simulink model "Lat_kinematics_Simul"  (R2022b)
settings: Solver=FixedStepAuto  StartTime=0.0  StopTime=tend  FixedStep=0.001  RelTol=1e-3
values from neighbouring files (symbols this model uses):
  lf = 1.4    [Lat_Dynamics_Simul_initialize.m]    (also in Lat_kinematics_Simul_initialize.m)
  lr = 1.6    [Lat_Dynamics_Simul_initialize.m]    (also in Lat_kinematics_Simul_initialize.m)
libraries: robotmobilelib x1
settings Model: Creator=LDW  LastModifiedBy=lego0

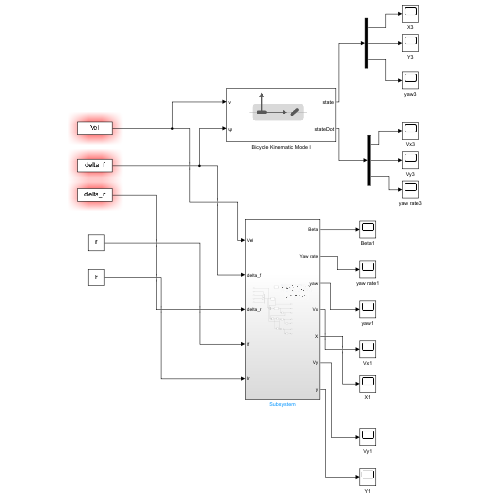
[thumbnail: Simulink's stored preview of the top-level diagram]
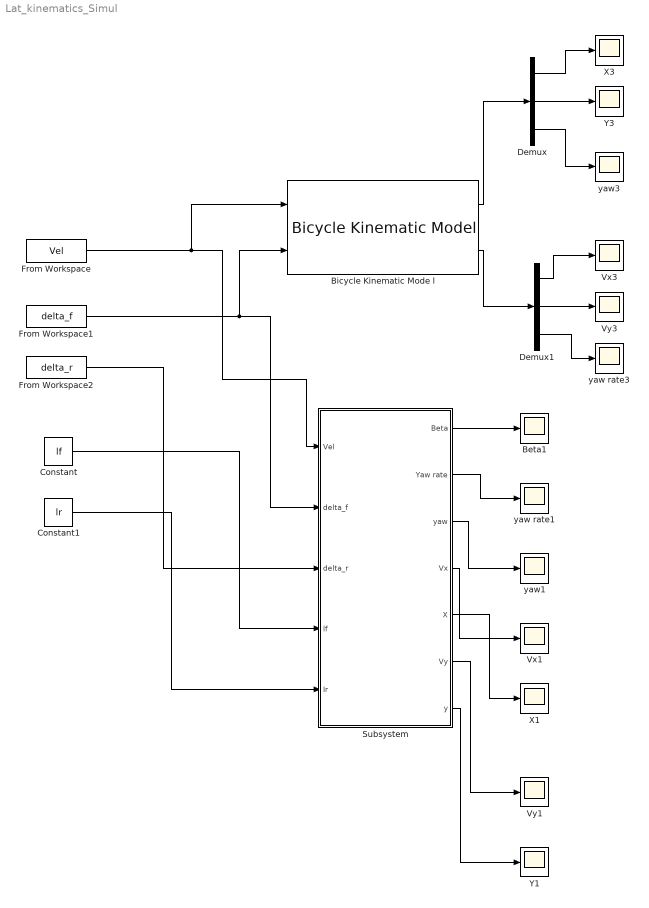
== system Lat_kinematics_Simul ==
  Beta1 : Scope
  Bicycle Kinematic Mode l : robotmobilelib/Bicycle Kinematic Model  VehicleInputs=Vehicle Speed & Steering Angle  WheelBase=3  VehicleSpeedRange=[-inf inf]  MaxSteeringAngle=pi/4  InitialState=[0; 0; 0]  SimulateUsing=Interpreted execution
  Constant : Constant  Value=lf
  Constant1 : Constant  Value=lr
  Demux : Demux  Outputs=3
  Demux1 : Demux  Outputs=3
  From Workspace : FromWorkspace  VariableName=Vel
  From Workspace1 : FromWorkspace  VariableName=delta_f
  From Workspace2 : FromWorkspace  VariableName=delta_r
  Subsystem : Subsystem
  Vx1 : Scope
  Vx3 : Scope
  Vy1 : Scope
  Vy3 : Scope
  X1 : Scope
  X3 : Scope
  Y1 : Scope
  Y3 : Scope
  yaw rate1 : Scope
  yaw rate3 : Scope
  yaw1 : Scope
  yaw3 : Scope
  wires:
  From Workspace/1 -> Subsystem/1(Vel), Bicycle Kinematic Mode l/1
  From Workspace1/1 -> Subsystem/2(delta_f), Bicycle Kinematic Mode l/2
  Bicycle Kinematic Mode l/1 -> Demux/1
  Bicycle Kinematic Mode l/2 -> Demux1/1
  Demux/3 -> yaw3/1
  Demux1/3 -> yaw rate3/1
  Demux1/2 -> Vy3/1
  Demux1/1 -> Vx3/1
  Demux/1 -> X3/1
  Demux/2 -> Y3/1
  From Workspace2/1 -> Subsystem/3(delta_r)
  Constant/1 -> Subsystem/4(lf)
  Constant1/1 -> Subsystem/5(Ir)
  Subsystem/1(Beta) -> Beta1/1
  Subsystem/2(Yaw rate) -> yaw rate1/1
  Subsystem/3(yaw) -> yaw1/1
  Subsystem/4(Vx) -> Vx1/1
  Subsystem/5(X) -> X1/1
  Subsystem/6(Vy) -> Vy1/1
  Subsystem/7(y) -> Y1/1

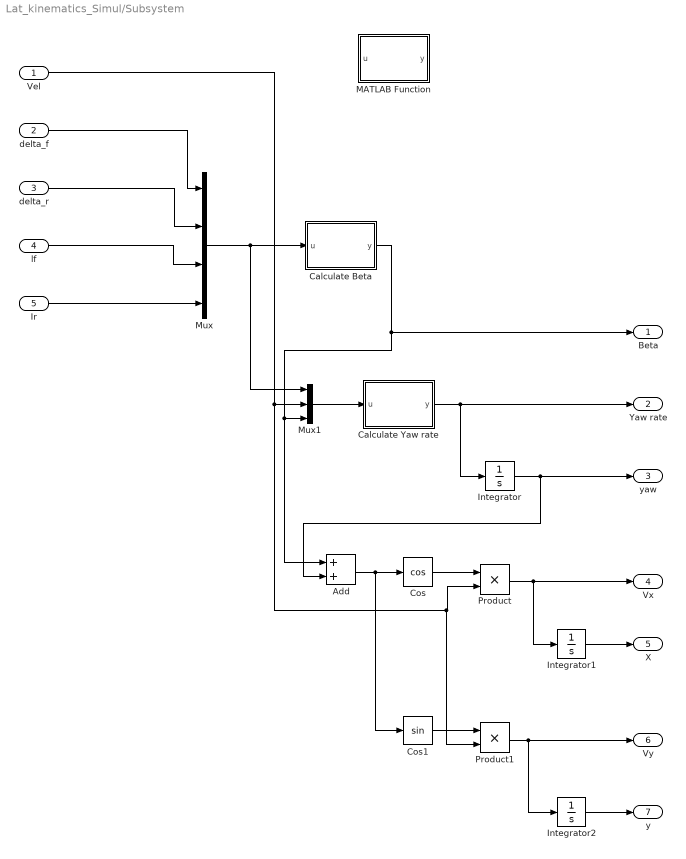
== system Lat_kinematics_Simul/Subsystem ==
  Vel : Inport
  delta_f : Inport  Port=2
  delta_r : Inport  Port=3
  lf : Inport  Port=4
  Ir : Inport  Port=5
  Add : Sum
  Calculate Beta : MATLAB Function  TreatAsAtomicUnit=on
  Calculate Yaw rate : MATLAB Function  TreatAsAtomicUnit=on
  Cos : Trigonometry  Operator=cos
  Cos1 : Trigonometry
  Integrator : Integrator
  Integrator1 : Integrator
  Integrator2 : Integrator
  "MATLAB Function " : MATLAB Function  TreatAsAtomicUnit=on
  Mux : Mux
  Mux1 : Mux  Inputs=3
  Product : Product
  Product1 : Product
  Beta : Outport
  Yaw rate : Outport  Port=2
  yaw : Outport  Port=3
  Vx : Outport  Port=4
  X : Outport  Port=5
  Vy : Outport  Port=6
  y : Outport  Port=7
  wires:
  Product/1 -> Vx/1, Integrator1/1
  Integrator/1 -> yaw/1, Add/2
  Add/1 -> Cos1/1, Cos/1
  Mux/1 -> Mux1/1, Calculate Beta/1(u)
  Calculate Yaw rate/1(y) -> Yaw rate/1, Integrator/1
  Cos/1 -> Product/1
  Vel/1 -> Product1/2, Product/2, Mux1/2
  Cos1/1 -> Product1/1
  Calculate Beta/1(y) -> Beta/1, Add/1, Mux1/3
  Product1/1 -> Vy/1, Integrator2/1
  Mux1/1 -> Calculate Yaw rate/1(u)
  Integrator2/1 -> y/1
  Ir/1 -> Mux/4
  delta_f/1 -> Mux/1
  lf/1 -> Mux/3
  delta_r/1 -> Mux/2
  Integrator1/1 -> X/1

== matlab function Lat_kinematics_Simul/Subsystem/Calculate Beta ==
  data: u input; y output
function y = fcn(u)

delta_f = u(1);
delta_r = u(2);
lf = u(3);
lr = u(4);

beta = atan((lf*tan(delta_r) + lr*tan(delta_f)) / (lf+lr));

y = beta;

== matlab function Lat_kinematics_Simul/Subsystem/MATLAB Function  ==
  data: u input; y output
function y = fcn(u)

y = u;

== matlab function Lat_kinematics_Simul/Subsystem/Calculate Yaw rate ==
  data: u input; y output
function y = fcn(u)

delta_f = u(1);
delta_r = u(2);
lf = u(3);
lr = u(4);
V = u(5);
beta = u(6);

yaw_rate = V*(tan(delta_f)+tan(delta_r))*cos(beta)/(lf+lr);

y = yaw_rate;
